simulink model "single_phase_afe_ideal"  (R2026a)
settings: Solver=ode23tb  StopTime=simlength  FixedStep=tc  MaxStep=glb_time.tc
values from neighbouring files (symbols this model uses):
  afe_ctrl = ctrl_afe_setup(glb_time.ts_afe, grid_emu.omega_grid_nom)    [init_model_legacy.m]
  frequency_set = 300    [init_model_legacy.m]
  glb_time = timing_setup(fpwm_afe, trgo_afe, fpwm_inv, trgo_inv, fpwm_single_phase_inv, trgo_single_phase_inv, fpwm_dab, trgo_dab,      fpwm_psfbc, trgo_psfbc, fpwm_isop_rail, trgo_isop_rail, fpwm_cllc, trgo_cllc, t_measure, tc_factor, tc_decimation, delay_pwm, dead_time_afe,      dead_time_inv, dead_time_single_phase_inv, dead_time_dab, dead_time_psfbc, dead_time_isop_rail, dead_time_cllc)    [init_model_legacy.m]
  grid_emu = grid_three_phase_emulator('Dyn11', delta_star, grid_nominal_power, application_voltage, us1, us2, fgrid,                  eq_grid_inductance, eq_grid_resistance, eta, ucc, i1m, p_iron, n1, n2, core_area, core_length, mur,                  up_xi_pu_ref, up_eta_pu_ref, un_xi_pu_ref, un_eta_pu_ref)    [init_model_legacy.m]
  heatsink = liquid_cooled_plate_2kw_setup(weight, no_weight, cp_al, heat_capacity_hs, thermal_conductivity_al,      Rth_switch_HA, Rth_mosfet_HA, Rth_diode_HA, Tambient, DThs_init)    [init_model_legacy.m]
  kepsilon = 2    [init_model_legacy.m]
  omega_set = frequency_set*2*pi    (= 1884.95559215)    [init_model_legacy.m]
  single_phase_inverter_ctrl = ctrl_single_phase_inverter_setup(glb_time.ts_inv, pres_ctrl.omega_set,      dqvector_pi.kp_inv, dqvector_pi.ki_inv, pres_ctrl.kp_rpi, pres_ctrl.ki_rpi, pres_ctrl.delta_rpi)    [init_model_legacy.m]
  Tambient = 40    [init_model_legacy.m]
  time_step_ref_1 = 0.025    [init_model_legacy.m]
  time_step_ref_2 = 0.5    [init_model_legacy.m]
  time_step_ref_3 = 1    [init_model_legacy.m]
  Vdc_nom = 400*1.35    (= 540)    [power_losses_calculation.m]
undefined symbols (not defined in the file or in its folder): delta_fht1, hwdata, igbt, Ld_fht1, magnitude, omega_fht1, ts_inv, Vac_FS, Xbez
libraries: fl_lib x116, nesl_utility x65, phase_shift_filter_ccaller x5, dq_vector_pi x4, igbt_simple_2th_lib x4, linear_double_integrator_observer_ccaller x3, lithium_ion_battery x1, dclink_for_two_levels x1, three_phase_voltage_with_frt_emulator x1, simulink x1, cstblocks_lti x1, single_phase_pwm_modulator x1
(part 3 of 6)

== system single_phase_afe_ideal/single_phase_inverter/single phase inverter control/single_phase_inverter_ctrl/dclink_ripple_compensation_dq/dq_vector_pi1/Subsystem ==
  x : Inport
  Gain1 : Gain  Gain=1/afe_ctrl.omega_base
  Terminator : Terminator
  linear_double_integrator_observer_ccaller : linear_double_integrator_observer_ccaller/linear_double_integrator_observer_ccaller  kx_m=afe_ctrl.di_obs.ktheta  kv_m=afe_ctrl.di_obs.komega  ts_m=glb_time.ts_afe  time_release=0.05  instance=2  tc_m=-1
  x_hat_ac : Outport
  wires:
  linear_double_integrator_observer_ccaller/2 -> Gain1/1
  linear_double_integrator_observer_ccaller/1 -> Terminator/1  "x_hat"
  x/1 -> linear_double_integrator_observer_ccaller/1
  Gain1/1 -> x_hat_ac/1  "x_hat_ac"

== system single_phase_afe_ideal/single_phase_inverter/single phase inverter control/single_phase_inverter_ctrl/dclink_ripple_compensation_dq/dq_vector_pi1/alphabeta2dq ==
  alpha : Inport
  beta : Inport  Port=2
  Gain : Gain  Gain=2
  MATLAB Function : MATLAB Function  TreatAsAtomicUnit=on
  "d " : Outport  VectorParamsAs1DForOutWhenUnconnected=off
  "q " : Outport  Port=2  VectorParamsAs1DForOutWhenUnconnected=off
  wires:
  alpha/1 -> MATLAB Function/1(alpha)
  beta/1 -> MATLAB Function/2(beta)
  MATLAB Function/1(d) -> "d "/1
  MATLAB Function/2(q) -> "q "/1
  [phase] -> Gain/1
  Gain/1 -> MATLAB Function/3(phase)

== system single_phase_afe_ideal/single_phase_inverter/single phase inverter control/single_phase_inverter_ctrl/dclink_ripple_compensation_dq/dq_vector_pi1/phase_shift_method_ccaller ==
  x_in : Inport
  Gain : Gain  Gain=-1
  phase_shift_filter_ccaller : phase_shift_filter_ccaller/phase_shift_filter_ccaller  freq_m=2*frequency_set  ts_m=glb_time.ts_inv  scaling_m=1  reset_time_release=0.025  instance=2  tc_m=-1
  x_out : Outport
  y_out : Outport  Port=2
  wires:
  phase_shift_filter_ccaller/1 -> Gain/1
  Gain/1 -> y_out/1  "y"
  x_in/1 -> x_out/1, phase_shift_filter_ccaller/1

== system single_phase_afe_ideal/single_phase_inverter/single phase inverter control/single_phase_inverter_ctrl/phase generator/FHT-PLL/pll_stageA ==
  gamma_grid : Inport
  ug_abc_pu : Inport  Port=2
  Demux : Demux  Outputs=3
  Math Function : Math  Operator=magnitude^2  SignedPower=on
  Math Function1 : Math  Operator=magnitude^2  SignedPower=on
  Reciprocal Sqrt : Sqrt  Operator=rSqrt
  Saturation : Saturate  UpperLimit=inf  LowerLimit=0.02
  Sum : Sum  Inputs=|++
  filter_and_transformation : Subsystem
  sequences : Subsystem
  u_grid_xi : Outport  VectorParamsAs1DForOutWhenUnconnected=off
  u_grid_eta : Outport  Port=2  VectorParamsAs1DForOutWhenUnconnected=off
  tag scope: Vgrid_unorm_fht=scoped
  wires:
  gamma_grid/1 -> sequences/3(phase_angle)
  sequences/2(u_grid_eta) -> u_grid_eta/1
  sequences/1(u_grid_xi) -> u_grid_xi/1
  ug_abc_pu/1 -> Demux/1
  Demux/1 -> filter_and_transformation/1(ug_a)
  Demux/2 -> filter_and_transformation/2(ug_b)
  Demux/3 -> filter_and_transformation/3(ug_c)
  filter_and_transformation/1(ug_alpha) -> Math Function/1, sequences/1(u_grid_alpha)
  filter_and_transformation/2(ug_beta) -> Math Function1/1, sequences/2(u_grid_beta)
  Math Function/1 -> Sum/1
  Math Function1/1 -> Sum/2
  Sum/1 -> Saturation/1
  Reciprocal Sqrt/1 -> [Vgrid_unorm_fht]
  Saturation/1 -> Reciprocal Sqrt/1

== system single_phase_afe_ideal/single_phase_inverter/single phase inverter control/single_phase_inverter_ctrl/phase generator/FHT-PLL/pll_stageB ==
  u_grid_pos_xi : Inport
  u_grid_pos_eta : Inport  Port=2
  Constant4 : Constant  Value=grid_emu.omega_grid_nom
  Gain : Gain  Gain=-1
  Product : Product  RndMeth=Zero
  Product1 : Product  RndMeth=Zero
  Product2 : Product  RndMeth=Zero
  Sum3 : Sum  SaturateOnIntegerOverflow=on
  Sum4 : Sum  SaturateOnIntegerOverflow=on
  Sum5 : Sum  Inputs=++|
  Terminator : Terminator
  Unit Delay1 : UnitDelay  SampleTime=-1
  Unit Delay2 : UnitDelay  SampleTime=-1
  Unit Delay4 : UnitDelay  SampleTime=-1
  bounder1 : MATLAB Function  TreatAsAtomicUnit=on
  double_integrator_observer : Subsystem
  kp : Gain  Gain=afe_ctrl.pll_i1_fht*glb_time.ts_afe  SaturateOnIntegerOverflow=on  OutDataTypeStr=Inherit: Same as input  ParamDataTypeStr=Inherit: Same as input
  kp1 : Gain  Gain=afe_ctrl.pll_p_fht  SaturateOnIntegerOverflow=on  OutDataTypeStr=Inherit: Same as input  ParamDataTypeStr=Inherit: Same as input
  kp2 : Gain  Gain=glb_time.ts_afe  SaturateOnIntegerOverflow=on  OutDataTypeStr=Inherit: Same as input  ParamDataTypeStr=Inherit: Same as input
  kp3 : Gain  Gain=1/grid_emu.omega_grid_nom  SaturateOnIntegerOverflow=on  OutDataTypeStr=Inherit: Same as input  ParamDataTypeStr=Inherit: Same as input
  gamma_grid_ddsrf_pll : Outport  VectorParamsAs1DForOutWhenUnconnected=off
  omega_grid_ddsrf_pll : Outport  Port=2  VectorParamsAs1DForOutWhenUnconnected=off
  wires:
  Gain/1 -> kp/1, kp1/1
  Product1/1 -> Gain/1
  kp3/1 -> omega_grid_ddsrf_pll/1
  Product/1 -> Terminator/1
  double_integrator_observer/1(omega_hat) -> kp3/1
  Unit Delay4/1 -> Sum3/2
  Sum4/1 -> bounder1/1(u)
  Unit Delay1/1 -> Sum4/2
  Sum3/1 -> Sum5/2, Unit Delay4/1  "i1"
  kp2/1 -> Sum4/1
  Constant4/1 -> Product2/2
  [Vgrid_unorm_fht] -> Product/2, Product1/2
  kp/1 -> Sum3/1
  Sum5/1 -> Product2/1
  bounder1/1(y) -> Unit Delay2/1, Unit Delay1/1
  u_grid_pos_xi/1 -> Product/1
  u_grid_pos_eta/1 -> Product1/1
  Product2/1 -> kp2/1
  kp1/1 -> Sum5/1
  Unit Delay2/1 -> double_integrator_observer/1(theta), gamma_grid_ddsrf_pll/1

== system single_phase_afe_ideal/single_phase_inverter/single phase inverter control/single_phase_inverter_ctrl/single_phase_current_control/dqpi_current_controller/alphabeta2dq ==
  alpha : Inport
  beta : Inport  Port=2
  MATLAB Function : MATLAB Function  TreatAsAtomicUnit=on
  "d " : Outport  VectorParamsAs1DForOutWhenUnconnected=off
  "q " : Outport  Port=2  VectorParamsAs1DForOutWhenUnconnected=off
  wires:
  alpha/1 -> MATLAB Function/1(alpha)
  beta/1 -> MATLAB Function/2(beta)
  MATLAB Function/1(d) -> "d "/1
  MATLAB Function/2(q) -> "q "/1
  [phase] -> MATLAB Function/3(phase)

== system single_phase_afe_ideal/single_phase_inverter/single phase inverter control/single_phase_inverter_ctrl/single_phase_current_control/dqpi_current_controller/dq2alphabeta ==
  d : Inport
  q : Inport  Port=2
  MATLAB Function : MATLAB Function  TreatAsAtomicUnit=on
  alpha : Outport  VectorParamsAs1DForOutWhenUnconnected=off
  wires:
  d/1 -> MATLAB Function/1(d)
  q/1 -> MATLAB Function/2(q)
  MATLAB Function/1(alpha) -> alpha/1
  [phase] -> MATLAB Function/3(phase)

== system single_phase_afe_ideal/single_phase_inverter/single phase inverter control/single_phase_inverter_ctrl/single_phase_current_control/dqpi_current_controller/dq_vector_pi ==
  id_ref : Inport
  id : Inport  Port=2
  iq : Inport  Port=3
  iq_ref : Inport  Port=4
  dq_vector_pi : dq_vector_pi/dq_vector_pi  kp=single_phase_inverter_ctrl.kp_inv  ki=single_phase_inverter_ctrl.ki_inv  ts=glb_time.ts_inv  lim_ctrl_out=single_phase_inverter_ctrl.u_lim  CTRPIFF_CLIP_RELEASE=CTRPIFF_CLIP_RELEASE
  ud_ctrl : Outport
  uq_ctrl : Outport  Port=2
  wires:
  id_ref/1 -> dq_vector_pi/1  "id_ref"
  iq_ref/1 -> dq_vector_pi/3  "iq_ref"
  dq_vector_pi/1 -> ud_ctrl/1  "ud_ctrl"
  iq/1 -> dq_vector_pi/4  "iq"
  id/1 -> dq_vector_pi/2  "id"
  dq_vector_pi/2 -> uq_ctrl/1  "uq_ctrl"
  [dclink_voltage_pu] -> dq_vector_pi/5

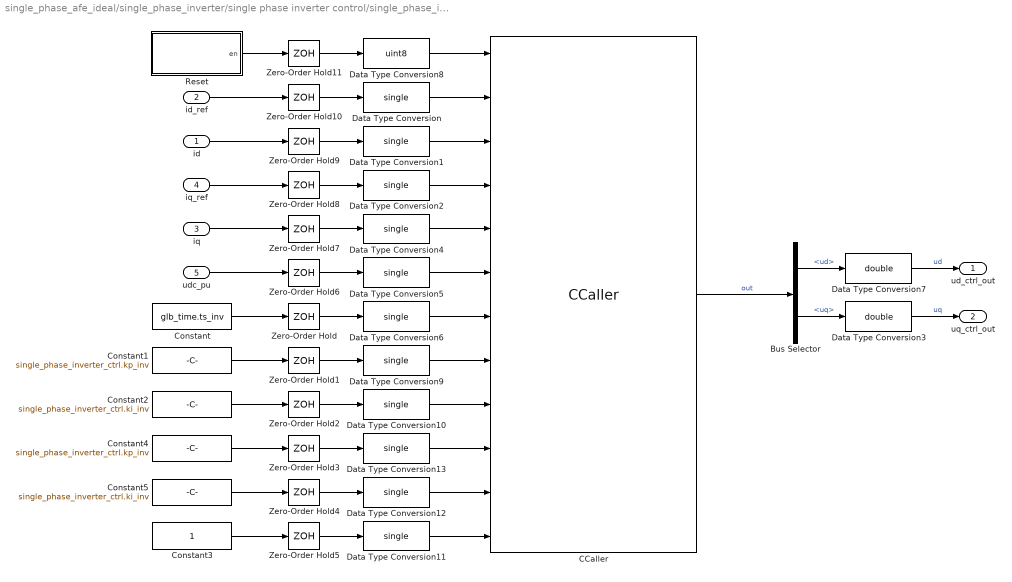
== system single_phase_afe_ideal/single_phase_inverter/single phase inverter control/single_phase_inverter_ctrl/single_phase_current_control/dqpi_current_controller/dq_vector_pi_ccaller ==
  id : Inport
  id_ref : Inport  Port=2
  iq : Inport  Port=3
  iq_ref : Inport  Port=4
  udc_pu : Inport  Port=5
  Bus Selector : BusSelector  OutputSignals=ud,uq
  CCaller : CCaller  FunctionName=dqvector_pi_process_simulink  PortSpecificationStruct="%)30     .    ,!8   8    (     @         %    \"     T    !     0         %  0 \"0    $    _    07)G3F%M90  4&]R=$YA;64 4V-O<&4     26YD97@     5'EP90      4VEZ90      27-';&]B86P   X    P    !@    @    $          4    (     0    ,    !         !   P!O=70 #@   #     &    \"     0         !0    @    !     P    $         $  # &]U=  .    .     8    (    !          %    \"     $    &     0         0   ...(+7280 chars)"
  Constant : Constant  Value=glb_time.ts_inv
  Constant1 : Constant  Value=single_phase_inverter_ctrl.kp_inv
  Constant2 : Constant  Value=single_phase_inverter_ctrl.ki_inv
  Constant3 : Constant
  Constant4 : Constant  Value=single_phase_inverter_ctrl.kp_inv
  Constant5 : Constant  Value=single_phase_inverter_ctrl.ki_inv
  Data Type Conversion{,1..2,4..6,9..13} (11 alike) : DataTypeConversion  OutDataTypeStr=single  SaturateOnIntegerOverflow=off  RndMeth=Floor
  Data Type Conversion3 : DataTypeConversion  OutDataTypeStr=double  SaturateOnIntegerOverflow=off  RndMeth=Floor
  Data Type Conversion7 : DataTypeConversion  OutDataTypeStr=double  SaturateOnIntegerOverflow=off  RndMeth=Floor
  Data Type Conversion8 : DataTypeConversion  OutDataTypeStr=uint8  SaturateOnIntegerOverflow=off  RndMeth=Floor
  Reset : Subsystem
  Zero-Order Hold{,1..11} (12 alike) : ZeroOrderHold  SampleTime=-1
  ud_ctrl_out : Outport
  uq_ctrl_out : Outport  Port=2
  wires:
  Data Type Conversion5/1 -> CCaller/6
  Data Type Conversion/1 -> CCaller/2
  CCaller/1 -> Bus Selector/1  "out"
  Data Type Conversion1/1 -> CCaller/3
  Data Type Conversion4/1 -> CCaller/5
  Data Type Conversion2/1 -> CCaller/4
  Data Type Conversion6/1 -> CCaller/7
  Bus Selector/2 -> Data Type Conversion3/1  "<uq>"
  Bus Selector/1 -> Data Type Conversion7/1  "<ud>"
  Data Type Conversion7/1 -> ud_ctrl_out/1  "ud"
  Data Type Conversion3/1 -> uq_ctrl_out/1  "uq"
  Data Type Conversion8/1 -> CCaller/1
  Data Type Conversion9/1 -> CCaller/8
  Data Type Conversion10/1 -> CCaller/9
  Data Type Conversion11/1 -> CCaller/12
  Data Type Conversion13/1 -> CCaller/10
  Data Type Conversion12/1 -> CCaller/11
  Constant3/1 -> Zero-Order Hold5/1
  Constant5/1 -> Zero-Order Hold4/1
  Constant4/1 -> Zero-Order Hold3/1
  Constant2/1 -> Zero-Order Hold2/1
  Constant1/1 -> Zero-Order Hold1/1
  Constant/1 -> Zero-Order Hold/1
  udc_pu/1 -> Zero-Order Hold6/1
  iq/1 -> Zero-Order Hold7/1
  iq_ref/1 -> Zero-Order Hold8/1
  Reset/1(en) -> Zero-Order Hold11/1
  id_ref/1 -> Zero-Order Hold10/1
  id/1 -> Zero-Order Hold9/1
  Zero-Order Hold/1 -> Data Type Conversion6/1
  Zero-Order Hold1/1 -> Data Type Conversion9/1
  Zero-Order Hold2/1 -> Data Type Conversion10/1
  Zero-Order Hold3/1 -> Data Type Conversion13/1
  Zero-Order Hold4/1 -> Data Type Conversion12/1
  Zero-Order Hold5/1 -> Data Type Conversion11/1
  Zero-Order Hold6/1 -> Data Type Conversion5/1
  Zero-Order Hold7/1 -> Data Type Conversion4/1
  Zero-Order Hold8/1 -> Data Type Conversion2/1
  Zero-Order Hold9/1 -> Data Type Conversion1/1
  Zero-Order Hold10/1 -> Data Type Conversion/1
  Zero-Order Hold11/1 -> Data Type Conversion8/1

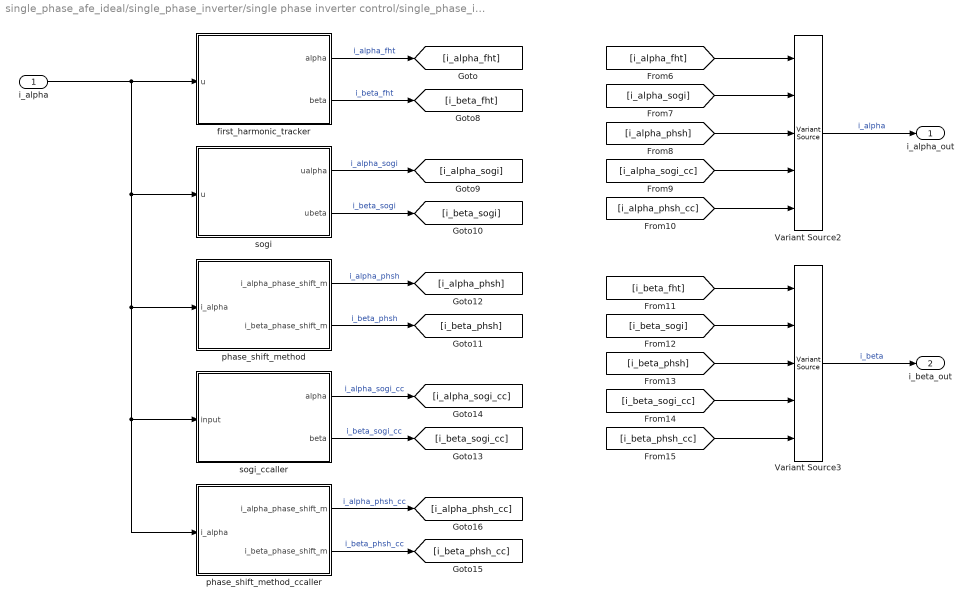
== system single_phase_afe_ideal/single_phase_inverter/single phase inverter control/single_phase_inverter_ctrl/single_phase_current_control/dqpi_current_controller/i2alphabeta ==
  i_alpha : Inport
  Variant Source2 : VariantSource  VariantControls="{use_single_phase_inverter_based_FHT == 1, use_single_phase_inverter_based_SOGI  == 1, use_single_phase_inverter_based_PHSH  == 1, use_single_phase_inverter_based_SOGI_ccaller  == 1, use_single_phase_inverter_based_PHSH_ccaller  == 1}"
  Variant Source3 : VariantSource  VariantControls="{use_single_phase_inverter_based_FHT == 1, use_single_phase_inverter_based_SOGI  == 1, use_single_phase_inverter_based_PHSH  == 1, use_single_phase_inverter_based_SOGI_ccaller  == 1, use_single_phase_inverter_based_PHSH_ccaller  == 1}"
  first_harmonic_tracker : Subsystem
  phase_shift_method : Subsystem
  phase_shift_method_ccaller : Subsystem
  sogi : Subsystem
  sogi_ccaller : Subsystem
  i_alpha_out : Outport
  i_beta_out : Outport  Port=2
  wires:
  i_alpha/1 -> phase_shift_method_ccaller/1(i_alpha), sogi_ccaller/1(input), phase_shift_method/1(i_alpha), sogi/1(u), first_harmonic_tracker/1(u)
  [i_alpha_phsh] -> Variant Source2/3
  [i_beta_sogi] -> Variant Source3/2
  [i_alpha_phsh_cc] -> Variant Source2/5
  first_harmonic_tracker/2(beta) -> [i_beta_fht]  "i_beta_fht"
  phase_shift_method/2(i_beta_phase_shift_m) -> [i_beta_phsh]  "i_beta_phsh"
  phase_shift_method/1(i_alpha_phase_shift_m) -> [i_alpha_phsh]  "i_alpha_phsh"
  [i_alpha_sogi] -> Variant Source2/2
  phase_shift_method_ccaller/1(i_alpha_phase_shift_m) -> [i_alpha_phsh_cc]  "i_alpha_phsh_cc"
  [i_beta_phsh_cc] -> Variant Source3/5
  [i_alpha_fht] -> Variant Source2/1
  [i_beta_phsh] -> Variant Source3/3
  sogi_ccaller/1(alpha) -> [i_alpha_sogi_cc]  "i_alpha_sogi_cc"
  [i_beta_sogi_cc] -> Variant Source3/4
  sogi/1(ualpha) -> [i_alpha_sogi]  "i_alpha_sogi"
  sogi/2(ubeta) -> [i_beta_sogi]  "i_beta_sogi"
  phase_shift_method_ccaller/2(i_beta_phase_shift_m) -> [i_beta_phsh_cc]  "i_beta_phsh_cc"
  sogi_ccaller/2(beta) -> [i_beta_sogi_cc]  "i_beta_sogi_cc"
  Variant Source2/1 -> i_alpha_out/1  "i_alpha"
  first_harmonic_tracker/1(alpha) -> [i_alpha_fht]  "i_alpha_fht"
  [i_alpha_sogi_cc] -> Variant Source2/4
  [i_beta_fht] -> Variant Source3/1
  Variant Source3/1 -> i_beta_out/1  "i_beta"

== system single_phase_afe_ideal/single_phase_inverter/single phase inverter control/single_phase_inverter_ctrl/sistem_identification/open loop u//f/dq2alphabeta ==
  Constant1 : Constant  Value=0
  Data Store Read : DataStoreRead  DataStoreName=u_test  IndexOptions=Index vector (dialog)  Indices=1  OutputSizes=1
  MATLAB Function : MATLAB Function  TreatAsAtomicUnit=on
  alpha : Outport  VectorParamsAs1DForOutWhenUnconnected=off
  wires:
  [phase] -> MATLAB Function/3(phase)
  MATLAB Function/1(alpha) -> alpha/1
  Data Store Read/1 -> MATLAB Function/1(d)
  Constant1/1 -> MATLAB Function/2(q)

== system single_phase_afe_ideal/single_phase_inverter/single phase inverter control/single_phase_inverter_ctrl/sistem_identification/open loop u//f/first_harmonic_tracker ==
  u : Inport
  Bus Selector : BusSelector  OutputSignals=output_pu_hat,output_pu_hat_dot
  Constant : Constant  Value=ts_inv
  Constant1 : Constant  Value=8
  Constant2 : Constant  Value=omega_fht1
  Constant3 : Constant  Value=delta_fht1
  Constant4 : Constant  Value=Ld_fht1(1)
  Constant5 : Constant  Value=Ld_fht1(2)
  Data Type Conversion{1..2,6..9} (6 alike) : DataTypeConversion  OutDataTypeStr=single  SaturateOnIntegerOverflow=off  RndMeth=Floor
  Data Type Conversion10 : DataTypeConversion  OutDataTypeStr=double  SaturateOnIntegerOverflow=off  RndMeth=Floor
  Data Type Conversion3 : DataTypeConversion  OutDataTypeStr=uint8  SaturateOnIntegerOverflow=off  RndMeth=Floor
  Data Type Conversion4 : DataTypeConversion  OutDataTypeStr=double  SaturateOnIntegerOverflow=off  RndMeth=Floor
  Data Type Conversion5 : DataTypeConversion  OutDataTypeStr=uint8  SaturateOnIntegerOverflow=off  RndMeth=Floor
  Gain : Gain  Gain=-1/omega_fht1
  Step : Step  Time=0.0125  InitialValue=1  FinalValue=0
  first_harmonic_tracker : CCaller  FunctionName=first_harmonic_tracker_process_simulink  PortSpecificationStruct="%)30     .    B \\   8    (     @         %    \"     D    !     0         %  0 \"0    $    _    07)G3F%M90  4&]R=$YA;64 4V-O<&4     26YD97@     5'EP90      4VEZ90      27-';&]B86P   X    P    !@    @    $          4    (     0    ,    !         !   P!O=70 #@   #     &    \"     0         !0    @    !     P    $         $  # &]U=  .    .     8    (    !          %    \"     $    &     0         0  ...(+4988 chars)"
  alpha : Outport
  beta : Outport  Port=2
  wires:
  Data Type Conversion4/1 -> alpha/1
  Data Type Conversion3/1 -> first_harmonic_tracker/1
  Data Type Conversion1/1 -> first_harmonic_tracker/3
  Data Type Conversion2/1 -> first_harmonic_tracker/2
  first_harmonic_tracker/1 -> Bus Selector/1
  Bus Selector/1 -> Data Type Conversion4/1  "<output_pu_hat>"
  Step/1 -> Data Type Conversion3/1
  u/1 -> Data Type Conversion2/1
  Constant/1 -> Data Type Conversion1/1
  Constant1/1 -> Data Type Conversion5/1
  Data Type Conversion5/1 -> first_harmonic_tracker/8
  Constant2/1 -> Data Type Conversion6/1
  Data Type Conversion6/1 -> first_harmonic_tracker/4
  Constant3/1 -> Data Type Conversion7/1
  Data Type Conversion7/1 -> first_harmonic_tracker/5
  Constant4/1 -> Data Type Conversion8/1
  Data Type Conversion8/1 -> first_harmonic_tracker/6
  Constant5/1 -> Data Type Conversion9/1
  Data Type Conversion9/1 -> first_harmonic_tracker/7
  Bus Selector/2 -> Data Type Conversion10/1  "<output_pu_hat_dot>"
  Data Type Conversion10/1 -> Gain/1
  Gain/1 -> beta/1

== system single_phase_afe_ideal/single_phase_inverter/single phase inverter control/single_phase_inverter_ctrl/sistem_identification/open loop u//f/module ==
  i_alpha : Inport
  i_beta : Inport  Port=2
  Sqrt : Sqrt
  Square : Math  Operator=square
  Square1 : Math  Operator=square
  Sum : Sum  Inputs=|++
  i : Outport
  wires:
  i_beta/1 -> Square1/1
  i_alpha/1 -> Square/1
  Square/1 -> Sum/1
  Sum/1 -> Sqrt/1
  Square1/1 -> Sum/2
  Sqrt/1 -> i/1  "i"

== system single_phase_afe_ideal/single_phase_inverter/single phase inverter control/single_phase_inverter_ctrl/sistem_identification/open loop u//f/sogi_ccaller ==
  input : Inport
  Bus Selector : BusSelector  OutputSignals=sogi_flt_output_alpha,sogi_flt_output_beta
  CCaller : CCaller  FunctionName=sogi_flt_process_simulink  PortSpecificationStruct="%)30     .    . P   8    (     @         %    \"     <    !     0         %  0 \"0    $    _    07)G3F%M90  4&]R=$YA;64 4V-O<&4     26YD97@     5'EP90      4VEZ90      27-';&]B86P   X    P    !@    @    $          4    (     0    ,    !         !   P!O=70 #@   #     &    \"     0         !0    @    !     P    $         $  # &]U=  .    .     8    (    !          %    \"     $    &     0         0   ...(+3829 chars)"
  Constant1 : Constant  Value=ts_inv
  Constant2 : Constant  Value=omega_set
  Constant3 : Constant  Value=kepsilon
  Constant4 : Constant  Value=0
  Data Type Conversion{1..2,4,6} (4 alike) : DataTypeConversion  OutDataTypeStr=single  SaturateOnIntegerOverflow=off  RndMeth=Floor
  Data Type Conversion3 : DataTypeConversion  OutDataTypeStr=uint8  SaturateOnIntegerOverflow=off  RndMeth=Floor
  Data Type Conversion5 : DataTypeConversion  OutDataTypeStr=double  SaturateOnIntegerOverflow=off  RndMeth=Floor
  Data Type Conversion7 : DataTypeConversion  OutDataTypeStr=double  SaturateOnIntegerOverflow=off  RndMeth=Floor
  Data Type Conversion8 : DataTypeConversion  OutDataTypeStr=uint8  SaturateOnIntegerOverflow=off  RndMeth=Floor
  Reset : Subsystem
  Zero-Order Hold{1..6} (6 alike) : ZeroOrderHold  SampleTime=-1
  alpha : Outport
  beta : Outport  Port=2
  wires:
  Zero-Order Hold6/1 -> Data Type Conversion4/1
  Data Type Conversion7/1 -> alpha/1
  Data Type Conversion4/1 -> CCaller/1
  Bus Selector/1 -> Data Type Conversion7/1  "<sogi_flt_output_alpha>"
  CCaller/1 -> Bus Selector/1
  Constant4/1 -> Zero-Order Hold5/1
  Zero-Order Hold5/1 -> Data Type Conversion3/1
  Constant2/1 -> Zero-Order Hold1/1
  Zero-Order Hold1/1 -> Data Type Conversion2/1
  Zero-Order Hold2/1 -> Data Type Conversion1/1
  Constant1/1 -> Zero-Order Hold2/1
  Reset/1(en) -> Zero-Order Hold4/1
  Zero-Order Hold4/1 -> Data Type Conversion8/1
  input/1 -> Zero-Order Hold6/1
  Bus Selector/2 -> Data Type Conversion5/1  "<sogi_flt_output_beta>"
  Data Type Conversion5/1 -> beta/1
  Data Type Conversion3/1 -> CCaller/6
  Data Type Conversion8/1 -> CCaller/5
  Data Type Conversion2/1 -> CCaller/3
  Data Type Conversion1/1 -> CCaller/2
  Data Type Conversion6/1 -> CCaller/4
  Zero-Order Hold3/1 -> Data Type Conversion6/1
  Constant3/1 -> Zero-Order Hold3/1

== system single_phase_afe_ideal/single_phase_inverter/single_phase_inverter/single phase inverter/three_phase_inverter_with_igbt_simple_2th/full_bridge_with_igbt_simple_2th/igbt_simple_1 ==
  note: P_sw
  Capacitor : fl_lib/Electrical/Electrical Elements/Capacitor  c=Csnubber_m F  r=Rsnubber_m Ohm  g=0 1/Ohm  i_specify=off  i_priority=None  i=0 A  i_nominal_specify=off  i_nominal_value=1  i_nominal_unit=A  v_specify=off  v_priority=None  v=0 V  v_nominal_specify=off  v_nominal_value=1  v_nominal_unit=V  vc_specify=off  vc_priority=High  vc=0 V  vc_nominal_specify=off  vc_nominal_value=1  vc_nominal_unit=V
  IGBT_simple : Subsystem
      settings: PortSchema="{\"entries\":[{\"content\":{\"sides\":[{\"content\":{\"connectorIds\":[\"LConn1\"]},\"type\":\"ConnectorPlacement.EquallySpacedRectSide\",\"uuid\":\"c3d88d60-081d-4221-ab18-079856838dba\"},{\"content\":{\"side\":\"RIGHT\"},\"type\":\"ConnectorPlacement.EquallySpacedRectSide\",\"uuid\":\"76e7d76c-8b60-4107-8aac-a7654bd886e1\"},{\"content\":{\"connectorIds\":[\"LConn2\"],\"side\":\"TOP\"},\"type\":\"ConnectorPlacement.EquallySpacedRectSide\",\"uuid\":\"fbef57e1-7143-4076-ada8-0654b1d9ee0b\"},{\"content\":{\"connectorIds\":[\"RConn1\"],\"side\":\"BOTTOM\"},\"type\":\"ConnectorPlacement.EquallySpacedRectSide\",\"uuid\":\"f2fea5db-9515-452a-a480-7d54bae36c49\"}]},\"type\":\"ConnectorPlacement.EquallySpacedConnector\",\"uuid\":\"cddff0b8-236e-4840-ad87-03abcdd65fe7\"}],\"packageUris\":[\"http://schema.mathworks.com/mf0/Connector/R2020b\"],\"version\":\"1.0\"}"
  Voltage Sensor : fl_lib/Electrical/Electrical Sensors/Voltage Sensor
  uph : nesl_utility/PS-Simulink Converter  PhysicalDomain=network_engine_domain  SubClassName=ps_output  LeftPortType=input  RightPortType=output  PseudoPeriodic=off  Frequencies=[]  VectorFormat=1-D array  Unit=V  AffineConversion=off
  G : PMIOPort  Side=Left
  C : PMIOPort  Port=2  Side=Left
  E : PMIOPort  Port=3  Side=Right
  tag scope: igbt_voltage_Q1=scoped
  wires:
  uph/1 -> [igbt_voltage_Q1]  "uph"
  connections:
  G/RConn1 -- IGBT_simple/LConn1
  Voltage Sensor/RConn1 -- uph/LConn1
  Capacitor/LConn1 -- Voltage Sensor/LConn1 -- C/RConn1 -- IGBT_simple/LConn2
  Capacitor/RConn1 -- Voltage Sensor/RConn2 -- E/RConn1 -- IGBT_simple/RConn1

== system single_phase_afe_ideal/single_phase_inverter/single_phase_inverter/single phase inverter/three_phase_inverter_with_igbt_simple_2th/full_bridge_with_igbt_simple_2th/igbt_simple_2 ==
  note: P_sw
  Capacitor : fl_lib/Electrical/Electrical Elements/Capacitor  c=Csnubber_m F  r=Rsnubber_m Ohm  g=0 1/Ohm  i_specify=off  i_priority=None  i=0 A  i_nominal_specify=off  i_nominal_value=1  i_nominal_unit=A  v_specify=off  v_priority=None  v=0 V  v_nominal_specify=off  v_nominal_value=1  v_nominal_unit=V  vc_specify=off  vc_priority=High  vc=0 V  vc_nominal_specify=off  vc_nominal_value=1  vc_nominal_unit=V
  IGBT_simple : Subsystem
      settings: PortSchema="{\"entries\":[{\"content\":{\"sides\":[{\"content\":{\"connectorIds\":[\"LConn1\"]},\"type\":\"ConnectorPlacement.EquallySpacedRectSide\",\"uuid\":\"c3d88d60-081d-4221-ab18-079856838dba\"},{\"content\":{\"side\":\"RIGHT\"},\"type\":\"ConnectorPlacement.EquallySpacedRectSide\",\"uuid\":\"76e7d76c-8b60-4107-8aac-a7654bd886e1\"},{\"content\":{\"connectorIds\":[\"LConn2\"],\"side\":\"TOP\"},\"type\":\"ConnectorPlacement.EquallySpacedRectSide\",\"uuid\":\"fbef57e1-7143-4076-ada8-0654b1d9ee0b\"},{\"content\":{\"connectorIds\":[\"RConn1\"],\"side\":\"BOTTOM\"},\"type\":\"ConnectorPlacement.EquallySpacedRectSide\",\"uuid\":\"f2fea5db-9515-452a-a480-7d54bae36c49\"}]},\"type\":\"ConnectorPlacement.EquallySpacedConnector\",\"uuid\":\"cddff0b8-236e-4840-ad87-03abcdd65fe7\"}],\"packageUris\":[\"http://schema.mathworks.com/mf0/Connector/R2020b\"],\"version\":\"1.0\"}"
  Voltage Sensor : fl_lib/Electrical/Electrical Sensors/Voltage Sensor
  uph : nesl_utility/PS-Simulink Converter  PhysicalDomain=network_engine_domain  SubClassName=ps_output  LeftPortType=input  RightPortType=output  PseudoPeriodic=off  Frequencies=[]  VectorFormat=1-D array  Unit=V  AffineConversion=off
  G : PMIOPort  Side=Left
  C : PMIOPort  Port=2  Side=Left
  E : PMIOPort  Port=3  Side=Right
  tag scope: igbt_voltage_Q2=scoped
  wires:
  uph/1 -> [igbt_voltage_Q2]  "uph"
  connections:
  IGBT_simple/RConn1 -- E/RConn1 -- Capacitor/RConn1 -- Voltage Sensor/RConn2
  C/RConn1 -- IGBT_simple/LConn2 -- Capacitor/LConn1 -- Voltage Sensor/LConn1
  Voltage Sensor/RConn1 -- uph/LConn1
  G/RConn1 -- IGBT_simple/LConn1

== system single_phase_afe_ideal/single_phase_inverter/single_phase_inverter/single phase inverter/three_phase_inverter_with_igbt_simple_2th/full_bridge_with_igbt_simple_2th/igbt_simple_3 ==
  note: P_sw
  Capacitor : fl_lib/Electrical/Electrical Elements/Capacitor  c=Csnubber_m F  r=Rsnubber_m Ohm  g=0 1/Ohm  i_specify=off  i_priority=None  i=0 A  i_nominal_specify=off  i_nominal_value=1  i_nominal_unit=A  v_specify=off  v_priority=None  v=0 V  v_nominal_specify=off  v_nominal_value=1  v_nominal_unit=V  vc_specify=off  vc_priority=High  vc=0 V  vc_nominal_specify=off  vc_nominal_value=1  vc_nominal_unit=V
  IGBT_simple : Subsystem
      settings: PortSchema="{\"entries\":[{\"content\":{\"sides\":[{\"content\":{\"connectorIds\":[\"LConn1\"]},\"type\":\"ConnectorPlacement.EquallySpacedRectSide\",\"uuid\":\"c3d88d60-081d-4221-ab18-079856838dba\"},{\"content\":{\"side\":\"RIGHT\"},\"type\":\"ConnectorPlacement.EquallySpacedRectSide\",\"uuid\":\"76e7d76c-8b60-4107-8aac-a7654bd886e1\"},{\"content\":{\"connectorIds\":[\"LConn2\"],\"side\":\"TOP\"},\"type\":\"ConnectorPlacement.EquallySpacedRectSide\",\"uuid\":\"fbef57e1-7143-4076-ada8-0654b1d9ee0b\"},{\"content\":{\"connectorIds\":[\"RConn1\"],\"side\":\"BOTTOM\"},\"type\":\"ConnectorPlacement.EquallySpacedRectSide\",\"uuid\":\"f2fea5db-9515-452a-a480-7d54bae36c49\"}]},\"type\":\"ConnectorPlacement.EquallySpacedConnector\",\"uuid\":\"cddff0b8-236e-4840-ad87-03abcdd65fe7\"}],\"packageUris\":[\"http://schema.mathworks.com/mf0/Connector/R2020b\"],\"version\":\"1.0\"}"
  Voltage Sensor : fl_lib/Electrical/Electrical Sensors/Voltage Sensor
  uph : nesl_utility/PS-Simulink Converter  PhysicalDomain=network_engine_domain  SubClassName=ps_output  LeftPortType=input  RightPortType=output  PseudoPeriodic=off  Frequencies=[]  VectorFormat=1-D array  Unit=V  AffineConversion=off
  G : PMIOPort  Side=Left
  C : PMIOPort  Port=2  Side=Left
  E : PMIOPort  Port=3  Side=Right
  tag scope: igbt_voltage_Q3=scoped
  wires:
  uph/1 -> [igbt_voltage_Q3]  "uph"
  connections:
  G/RConn1 -- IGBT_simple/LConn1
  Voltage Sensor/RConn1 -- uph/LConn1
  Voltage Sensor/LConn1 -- Capacitor/LConn1 -- IGBT_simple/LConn2 -- C/RConn1
  Voltage Sensor/RConn2 -- Capacitor/RConn1 -- E/RConn1 -- IGBT_simple/RConn1

== system single_phase_afe_ideal/single_phase_inverter/single_phase_inverter/single phase inverter/three_phase_inverter_with_igbt_simple_2th/full_bridge_with_igbt_simple_2th/igbt_simple_4 ==
  note: P_sw
  Capacitor : fl_lib/Electrical/Electrical Elements/Capacitor  c=Csnubber_m F  r=Rsnubber_m Ohm  g=0 1/Ohm  i_specify=off  i_priority=None  i=0 A  i_nominal_specify=off  i_nominal_value=1  i_nominal_unit=A  v_specify=off  v_priority=None  v=0 V  v_nominal_specify=off  v_nominal_value=1  v_nominal_unit=V  vc_specify=off  vc_priority=High  vc=0 V  vc_nominal_specify=off  vc_nominal_value=1  vc_nominal_unit=V
  IGBT_simple : Subsystem
      settings: PortSchema="{\"entries\":[{\"content\":{\"sides\":[{\"content\":{\"connectorIds\":[\"LConn1\"]},\"type\":\"ConnectorPlacement.EquallySpacedRectSide\",\"uuid\":\"c3d88d60-081d-4221-ab18-079856838dba\"},{\"content\":{\"side\":\"RIGHT\"},\"type\":\"ConnectorPlacement.EquallySpacedRectSide\",\"uuid\":\"76e7d76c-8b60-4107-8aac-a7654bd886e1\"},{\"content\":{\"connectorIds\":[\"LConn2\"],\"side\":\"TOP\"},\"type\":\"ConnectorPlacement.EquallySpacedRectSide\",\"uuid\":\"fbef57e1-7143-4076-ada8-0654b1d9ee0b\"},{\"content\":{\"connectorIds\":[\"RConn1\"],\"side\":\"BOTTOM\"},\"type\":\"ConnectorPlacement.EquallySpacedRectSide\",\"uuid\":\"f2fea5db-9515-452a-a480-7d54bae36c49\"}]},\"type\":\"ConnectorPlacement.EquallySpacedConnector\",\"uuid\":\"cddff0b8-236e-4840-ad87-03abcdd65fe7\"}],\"packageUris\":[\"http://schema.mathworks.com/mf0/Connector/R2020b\"],\"version\":\"1.0\"}"
  Voltage Sensor : fl_lib/Electrical/Electrical Sensors/Voltage Sensor
  uph : nesl_utility/PS-Simulink Converter  PhysicalDomain=network_engine_domain  SubClassName=ps_output  LeftPortType=input  RightPortType=output  PseudoPeriodic=off  Frequencies=[]  VectorFormat=1-D array  Unit=V  AffineConversion=off
  G : PMIOPort  Side=Left
  C : PMIOPort  Port=2  Side=Left
  E : PMIOPort  Port=3  Side=Right
  tag scope: igbt_voltage_Q4=scoped
  wires:
  uph/1 -> [igbt_voltage_Q4]  "uph"
  connections:
  IGBT_simple/RConn1 -- E/RConn1 -- Capacitor/RConn1 -- Voltage Sensor/RConn2
  C/RConn1 -- IGBT_simple/LConn2 -- Capacitor/LConn1 -- Voltage Sensor/LConn1
  Voltage Sensor/RConn1 -- uph/LConn1
  G/RConn1 -- IGBT_simple/LConn1

== system single_phase_afe_ideal/single_phase_inverter/single_phase_inverter/single phase inverter/three_phase_inverter_with_igbt_simple_2th/full_bridge_with_igbt_simple_2th/module_1 ==
  Bus Creator : BusCreator  Inputs=18
  m : Outport
  wires:
  [diode_HA_temp_Q1] -> Bus Creator/8  "diode_HA_temp_Q1"
  [igbt_voltage_Q2] -> Bus Creator/10  "igbt_voltage_Q2"
  [igbt_voltage_Q1] -> Bus Creator/2  "igbt_voltage_Q1"
  [igbt_ploss_Q2] -> Bus Creator/9  "igbt_ploss_Q2"
  [igbt_current_Q2] -> Bus Creator/11  "igbt_current_Q2"
  [diode_ploss_Q1] -> Bus Creator/6  "diode_ploss_Q1"
  [diode_JH_temp_Q1] -> Bus Creator/7  "diode_JH_temp_Q1"
  [igbt_HA_temp_Q1] -> Bus Creator/5  "igbt_HA_temp_Q1"
  [igbt_ploss_Q1] -> Bus Creator/1  "igbt_ploss_Q1"
  [diode_JH_temp_Q2] -> Bus Creator/15  "diode_JH_temp_Q2"
  [diode_HA_temp_Q2] -> Bus Creator/16  "diode_HA_temp_Q2"
  [diode_ploss_Q2] -> Bus Creator/14  "diode_ploss_Q2"
  [igbt_HA_temp_Q2] -> Bus Creator/13  "igbt_HA_temp_Q2"
  [igbt_JH_temp_Q2] -> Bus Creator/12  "igbt_JH_temp_Q2"
  [igbt_JH_temp_Q1] -> Bus Creator/4  "igbt_JH_temp_Q1"
  [igbt_current_Q1] -> Bus Creator/3  "igbt_current_Q1"
  Bus Creator/1 -> m/1  "module_1"
  [diode_current_Q1] -> Bus Creator/17  "diode_current_Q1"
  [diode_current_Q2] -> Bus Creator/18  "diode_current_Q2"

== system single_phase_afe_ideal/single_phase_inverter/single_phase_inverter/single phase inverter/three_phase_inverter_with_igbt_simple_2th/full_bridge_with_igbt_simple_2th/module_2 ==
  Bus Creator1 : BusCreator  Inputs=18
  m : Outport
  wires:
  [diode_HA_temp_Q4] -> Bus Creator1/16  "diode_HA_temp_Q4"
  [igbt_HA_temp_Q3] -> Bus Creator1/5  "igbt_HA_temp_Q3"
  [igbt_JH_temp_Q3] -> Bus Creator1/4  "igbt_JH_temp_Q3"
  [diode_ploss_Q3] -> Bus Creator1/6  "diode_ploss_Q3"
  [diode_JH_temp_Q4] -> Bus Creator1/15  "diode_JH_temp_Q4"
  [igbt_ploss_Q3] -> Bus Creator1/1  "igbt_ploss_Q3"
  [igbt_JH_temp_Q4] -> Bus Creator1/12  "igbt_JH_temp_Q4"
  [igbt_voltage_Q3] -> Bus Creator1/2  "igbt_voltage_Q3"
  [igbt_current_Q4] -> Bus Creator1/11  "igbt_current_Q4"
  [diode_HA_temp_Q3] -> Bus Creator1/8  "diode_HA_temp_Q3"
  [igbt_voltage_Q4] -> Bus Creator1/10  "igbt_voltage_Q4"
  [igbt_ploss_Q4] -> Bus Creator1/9  "igbt_ploss_Q4"
  [igbt_HA_temp_Q4] -> Bus Creator1/13  "igbt_HA_temp_Q4"
  [diode_JH_temp_Q3] -> Bus Creator1/7  "diode_JH_temp_Q3"
  [diode_ploss_Q4] -> Bus Creator1/14  "diode_ploss_Q4"
  [igbt_current_Q3] -> Bus Creator1/3  "igbt_current_Q3"
  Bus Creator1/1 -> m/1  "module_2"
  [diode_current_Q4] -> Bus Creator1/18  "diode_current_Q4"
  [diode_current_Q3] -> Bus Creator1/17  "diode_current_Q3"
